simulink model "ackermannbizhang"  (R2026a)
settings: Solver=VariableStepAuto
undefined symbols (not defined in the file or in its folder): radarD, radarX
libraries: robotmobilelib x1, simulink x1
settings Model: Creator=hanjiatong  LastModifiedBy=hanjiatong

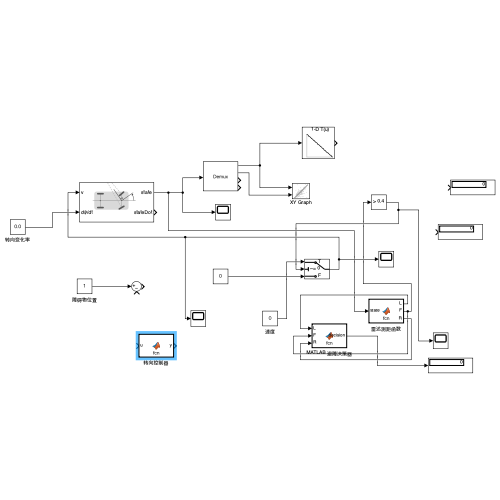
[thumbnail: Simulink's stored preview of the top-level diagram]
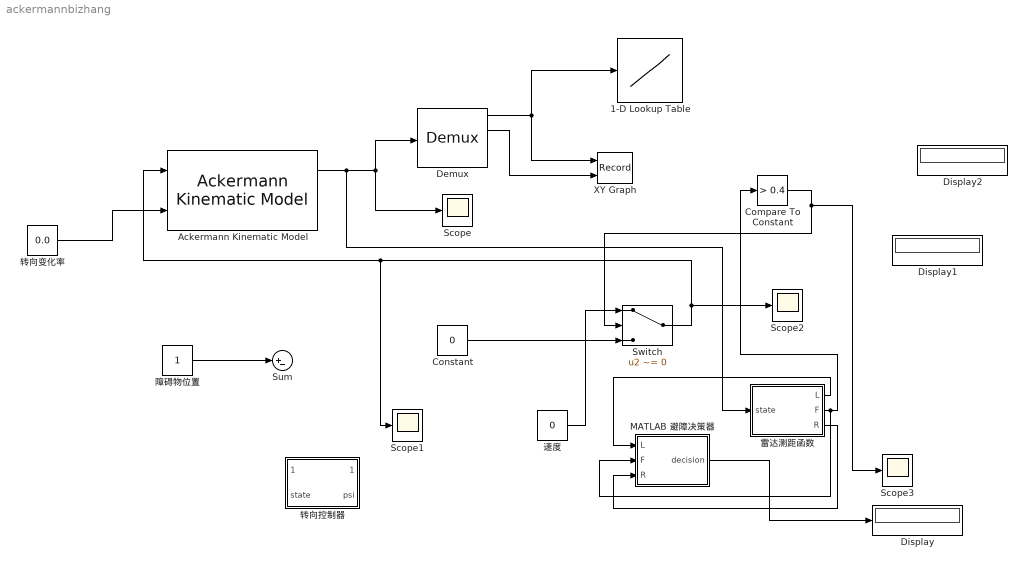
== system ackermannbizhang ==
  1-D Lookup Table : Lookup_n-D  NumberOfTableDimensions=1  BreakpointsForDimension1=radarX  Table=radarD  ExtrapMethod=Clip  InternalRulePriority=Speed  RndMeth=Simplest
  Ackermann Kinematic Model : robotmobilelib/Ackermann Kinematic Model  WheelBase=0.144  VehicleSpeedRange=[-inf inf]  MaxSteeringAngle=pi/4  InitialState=[0.5; 1.5; 0; 0]  SimulateUsing=Interpreted execution
  Compare To Constant : simulink/Logic and Bit Operations/Compare To Constant  relop=>  const=0.4  OutDataTypeStr=boolean
  Constant : Constant  Value=0
  Demux : Demux
      settings: DisplayOption=none
  Display : Display
  Display1 : Display
  Display2 : Display
  MATLAB 避障决策器 : MATLAB Function  TreatAsAtomicUnit=on
  Scope{,1..3} (4 alike) : Scope
      Scope settings: ActiveDisplayYMinimum=-0.19594221664657985  ActiveDisplayYMaximum=1.7514452129987257
      Scope1 settings: ActiveDisplayYMinimum=-1  ActiveDisplayYMaximum=1
      Scope2 settings: ActiveDisplayYMinimum=-0.018749999999999996  ActiveDisplayYMaximum=0.16874999999999998  DataLoggingVariableName=ScopeData2
      Scope3 settings: ActiveDisplayYMinimum=0.33124999999999571  ActiveDisplayYMaximum=1.018749999999998  DataLoggingVariableName=ScopeData3
  Sum : Sum  Inputs=|+-
  Switch : Switch  Criteria=u2 ~= 0  SaturateOnIntegerOverflow=off  InputSameDT=off
  XY Graph : Record  NumPorts=2.0  FileSettingsInternal="{\"entries\":[{\"content\":{\"excelSettings\":{\"content\":{},\"type\":\"Streamout.ExcelSettings\"},\"parquetSettings\":{\"content\":{},\"type\":\"Streamout.ParquetSettings\"}},\"type\":\"Streamout.FileSettingStorage\",\"uuid\":\"\"}],\"packageUris\":[\"http:\\/\\/schema.mathworks.com\\/mf0\\/streamout_blocks\\/R2020a\"],\"version\":\"1.0\"}"  FrameSettings=[0, 0]  Layout=[1 1]  SignalsInternal="{\"entries\":[{\"content\":{\"signals\":[{\"content\":{\"blockPath\":[],\"dimensions\":[1],\"domain\":\"\",\"lineColor\":\"#a2142f\",\"plots\":[ 1 ],\"port\":1,\"sid\":[\"\"],\"signalID\":1,\"signalName\":\"Demux:1\"},\"type\":\"RecordBlkView.Signal\",\"uuid\":\"\"},{\"content\":{\"blockPath\":[],\"dimensions\":[1],\"domain\":\"\",\"lineColor\":\"#139fff\",\"plots\":[ 1 ],\"port\":2,\"sid\":[\"\"],\"signalID\":2,\"signalName\":\"Demux:2\"},\"type\":\"RecordBlkView.Signal\",\"uuid\":\"\"}]},\"type\":\"RecordBlkView.InputSignals\",\"uuid\":\"\"}],\"packageUris\":[\"http:\\/\\/schema.mathworks.com\\/mf0\\/streamout_blocks\\/R2020a\"],\"version\":\"1.0\"}"  VisualizationBindings="{\"xyplotplugin\":{\"info\":[{\"series\":[{\"bindingParametersList\":[{\"parameter\":\"X-Axis\",\"signalID\":1,\"signalName\":\"Demux:1\"},{\"parameter\":\"Y-Axis\",\"signalID\":2,\"signalName\":\"Demux:2\"}],\"seriesID\":0}],\"subplotID\":1}]}}"  CompatibilityTag=XY
  转向变化率 : Constant  Value=0.0
  转向控制器 : MATLAB Function  TreatAsAtomicUnit=on
  速度 : Constant  Value=0
  障碍物位置 : Constant
  雷达测距函数 : MATLAB Function  TreatAsAtomicUnit=on
  wires:
  转向变化率/1 -> Ackermann Kinematic Model/2
  Ackermann Kinematic Model/1 -> 雷达测距函数/1(state), Scope/1, Demux/1
  Demux/1 -> XY Graph/1, 1-D Lookup Table/1
  Demux/2 -> XY Graph/2
  障碍物位置/1 -> Sum/1
  Switch/1 -> Scope2/1, Scope1/1, Ackermann Kinematic Model/1
  Compare To Constant/1 -> Scope3/1, Switch/2
  速度/1 -> Switch/1
  Constant/1 -> Switch/3
  雷达测距函数/2(F) -> MATLAB 避障决策器/2(F), Compare To Constant/1
  雷达测距函数/1(L) -> MATLAB 避障决策器/1(L)
  雷达测距函数/3(R) -> MATLAB 避障决策器/3(R)
  MATLAB 避障决策器/1(decision) -> Display/1

== matlab function ackermannbizhang/雷达测距函数 ==
  data: state input; L output; F output; R output

function [L, F, R] = fcn(state)
% 输入：小车的状态
% 输出：左、前、右三个方向的障碍物距离

% 在 MATLAB 中执行我们的雷达测距函数
coder.extrinsic('l150ThreeRanges');

% 获取小车的实时位置和朝向
x = state(1);
y = state(2);
theta = state(3);

pose = [x, y, theta];

% 预先声明三个输出都是数值
L = 3.0;
F = 3.0;
R = 3.0;

% 调用刚才写好的三方向雷达函数
[L, F, R] = l150ThreeRanges(pose);

end

== matlab function ackermannbizhang/转向控制器 ==
  data: decision input; psiRate output; state input; psi output

function [psiRate, psi] = fcn(decision, state)
% 根据避障决定控制前轮转向

% 读取当前前轮转角
psi = state(4);

% 设定目标转角
if decision == 2
    psiTarget = 0.15;    % 左转
elseif decision == 3
    psiTarget = -0.15;   % 右转
else
    psiTarget = 0;       % 回正
end

% 根据转角误差计算转向变化率
error = psiTarget - psi;
psiRate = 2 * error;

% 限制转向速度
psiRate = max(-0.1, min(0.1, psiRate));

end

== matlab function ackermannbizhang/MATLAB 避障决策器 ==
  data: L input; decision output; F input; R input

function decision = fcn(L, F, R)
% 避障决策器
% 0 = 前方畅通
% 1 = 停车，暂时无法确定安全绕行方向
% 2 = 左侧可以考虑绕行
% 3 = 右侧可以考虑绕行

decision = 1;

% 前方距离足够远
if F > 0.6
    decision = 0;

% 前方存在需要处理的障碍物
elseif L > 0.8 && L > R + 0.1
    decision = 2;

elseif R > 0.8 && R > L + 0.1
    decision = 3;

else
    decision = 1;
end

end
